simulink model "OpenLoop_TraditionalStepper"  (R2026a)
settings: Solver=FixedStepDiscrete  StopTime=0.05  FixedStep=Ts_sim
undefined symbols (not defined in the file): adc_counts_at_zero_current, amps_per_adc_count, number_of_steps_to_move, phase_voltage_volts, sequence_start_angle_radians, step_angle_radians, step_direction, step_rate_steps_per_second, step_sequence_phase_a, step_sequence_phase_b, steps_in_sequence, Ts_sim
settings Model: Creator=drew  LastModifiedBy=Drew

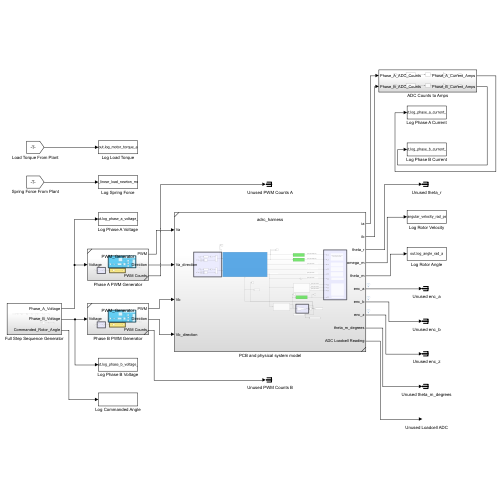
[thumbnail: Simulink's stored preview of the top-level diagram]
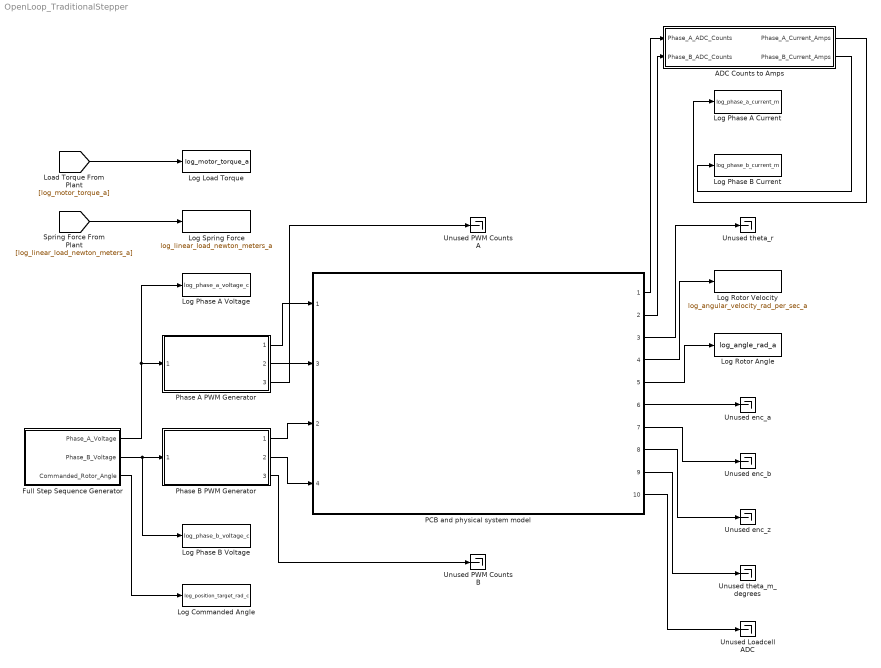
== system OpenLoop_TraditionalStepper ==
  ADC Counts to Amps : Subsystem
  Full Step Sequence Generator : Subsystem
  Log Commanded Angle : ToWorkspace  VariableName=log_position_target_rad_c  SaveFormat=Timeseries  SampleTime=-1
      settings: Decimation=logging_decimation
  Log Load Torque : ToWorkspace  VariableName=log_motor_torque_a  SaveFormat=Timeseries  SampleTime=-1
      settings: Decimation=logging_decimation
  Log Phase A Current : ToWorkspace  VariableName=log_phase_a_current_m  SaveFormat=Timeseries  SampleTime=-1
      settings: Decimation=logging_decimation
  Log Phase A Voltage : ToWorkspace  VariableName=log_phase_a_voltage_c  SaveFormat=Timeseries  SampleTime=-1
      settings: Decimation=logging_decimation
  Log Phase B Current : ToWorkspace  VariableName=log_phase_b_current_m  SaveFormat=Timeseries  SampleTime=-1
      settings: Decimation=logging_decimation
  Log Phase B Voltage : ToWorkspace  VariableName=log_phase_b_voltage_c  SaveFormat=Timeseries  SampleTime=-1
      settings: Decimation=logging_decimation
  Log Rotor Angle : ToWorkspace  VariableName=log_angle_rad_a  SaveFormat=Timeseries  SampleTime=-1
      settings: Decimation=logging_decimation
  Log Rotor Velocity : ToWorkspace  VariableName=log_angular_velocity_rad_per_sec_a  SaveFormat=Timeseries  SampleTime=-1
      settings: Decimation=logging_decimation
  Log Spring Force : ToWorkspace  VariableName=log_linear_load_newton_meters_a  SaveFormat=Timeseries  SampleTime=-1
      settings: Decimation=logging_decimation
  PCB and physical system model : Subsystem  ReferencedSubsystem=adrc_harness
      settings: PortSchema="{\"entries\":[{\"content\":{\"sides\":[{\"content\":{\"connectorIds\":[\"In1\",\"In3\",\"In2\",\"In4\"]},\"type\":\"ConnectorPlacement.EquallySpacedRectSide\",\"uuid\":\"db952c66-fc57-447a-862c-b79330cada38\"},{\"content\":{\"connectorIds\":[\"Out1\",\"Out2\",\"Out3\",\"Out4\",\"Out5\",\"Out6\",\"Out7\",\"Out8\",\"Out9\",\"Out10\"],\"side\":\"RIGHT\"},\"type\":\"ConnectorPlacement.EquallySpacedRectSide\",\"uuid\":\"12562dc1-b5c4-4239-b729-963395de8428\"},{\"content\":{\"side\":\"TOP\"},\"type\":\"ConnectorPlacement.EquallySpacedRectSide\",\"uuid\":\"3dbdfbee-8cdb-483e-891a-ab3c030ef055\"}]},\"type\":\"ConnectorPlacement.EquallySpacedConnector\",\"uuid\":\"9d79cb43-5fdf-4c5b-b972-7a6fb554b8ba\"}],\"packageUris\":[\"http://schema.mathworks.com/mf0/Connector/R2020b\"],\"version\":\"1.0\"}"
  Phase A PWM Generator : Subsystem  ReferencedSubsystem=PWM_Generator
  Phase B PWM Generator : Subsystem  ReferencedSubsystem=PWM_Generator
  Unused Loadcell ADC : Terminator
  Unused PWM Counts A : Terminator
  Unused PWM Counts B : Terminator
  Unused enc_a : Terminator
  Unused enc_b : Terminator
  Unused enc_z : Terminator
  Unused theta_m_degrees : Terminator
  Unused theta_r : Terminator
  wires:
  Phase B PWM Generator/3 -> Unused PWM Counts B/1
  Phase A PWM Generator/3 -> Unused PWM Counts A/1
  PCB and physical system model/10 -> Unused Loadcell ADC/1
  PCB and physical system model/9 -> Unused theta_m_degrees/1
  PCB and physical system model/8 -> Unused enc_z/1
  PCB and physical system model/7 -> Unused enc_b/1
  PCB and physical system model/6 -> Unused enc_a/1
  PCB and physical system model/3 -> Unused theta_r/1
  [log_linear_load_newton_meters_a] -> Log Spring Force/1
  [log_motor_torque_a] -> Log Load Torque/1
  PCB and physical system model/5 -> Log Rotor Angle/1
  PCB and physical system model/4 -> Log Rotor Velocity/1
  Full Step Sequence Generator/3(Commanded_Rotor_Angle) -> Log Commanded Angle/1
  Full Step Sequence Generator/1(Phase_A_Voltage) -> Phase A PWM Generator/1, Log Phase A Voltage/1
  Full Step Sequence Generator/2(Phase_B_Voltage) -> Phase B PWM Generator/1, Log Phase B Voltage/1
  Phase B PWM Generator/2 -> PCB and physical system model/4
  Phase B PWM Generator/1 -> PCB and physical system model/2
  Phase A PWM Generator/2 -> PCB and physical system model/3
  Phase A PWM Generator/1 -> PCB and physical system model/1
  ADC Counts to Amps/2(Phase_B_Current_Amps) -> Log Phase B Current/1
  ADC Counts to Amps/1(Phase_A_Current_Amps) -> Log Phase A Current/1
  PCB and physical system model/1 -> ADC Counts to Amps/1(Phase_A_ADC_Counts)
  PCB and physical system model/2 -> ADC Counts to Amps/2(Phase_B_ADC_Counts)

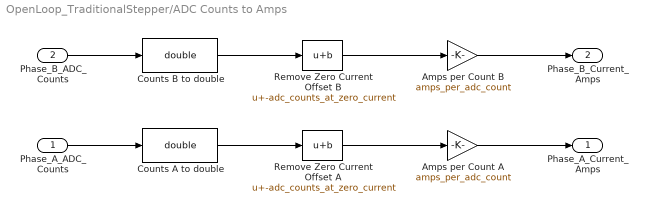
== system OpenLoop_TraditionalStepper/ADC Counts to Amps ==
  Phase_A_ADC_Counts : Inport
  Phase_B_ADC_Counts : Inport  Port=2
  Amps per Count A : Gain  Gain=amps_per_adc_count
  Amps per Count B : Gain  Gain=amps_per_adc_count
  Counts A to double : DataTypeConversion  OutDataTypeStr=double  SaturateOnIntegerOverflow=off  RndMeth=Floor
  Counts B to double : DataTypeConversion  OutDataTypeStr=double  SaturateOnIntegerOverflow=off  RndMeth=Floor
  Remove Zero Current Offset A : Bias  Bias=-adc_counts_at_zero_current  SaturateOnIntegerOverflow=off
  Remove Zero Current Offset B : Bias  Bias=-adc_counts_at_zero_current  SaturateOnIntegerOverflow=off
  Phase_A_Current_Amps : Outport
  Phase_B_Current_Amps : Outport  Port=2
  wires:
  Amps per Count B/1 -> Phase_B_Current_Amps/1
  Remove Zero Current Offset B/1 -> Amps per Count B/1
  Counts B to double/1 -> Remove Zero Current Offset B/1
  Phase_B_ADC_Counts/1 -> Counts B to double/1
  Amps per Count A/1 -> Phase_A_Current_Amps/1
  Remove Zero Current Offset A/1 -> Amps per Count A/1
  Counts A to double/1 -> Remove Zero Current Offset A/1
  Phase_A_ADC_Counts/1 -> Counts A to double/1

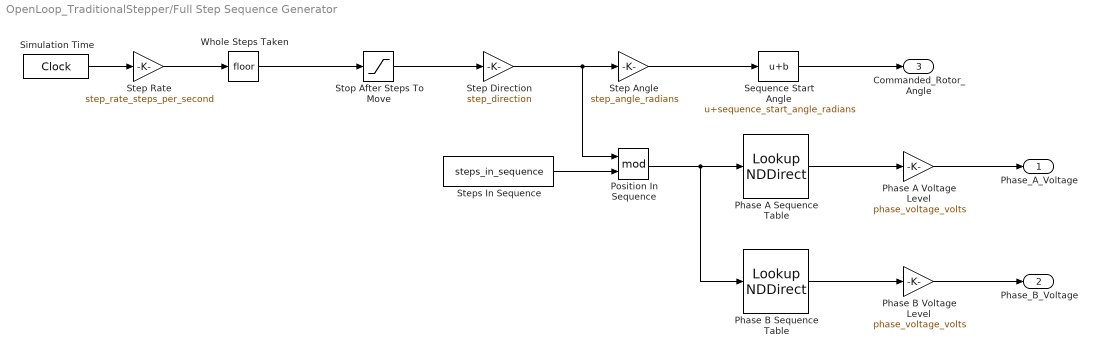
== system OpenLoop_TraditionalStepper/Full Step Sequence Generator ==
  Phase A Sequence Table : LookupNDDirect  NumberOfTableDimensions=1  Table=step_sequence_phase_a
  Phase A Voltage Level : Gain  Gain=phase_voltage_volts
  Phase B Sequence Table : LookupNDDirect  NumberOfTableDimensions=1  Table=step_sequence_phase_b
  Phase B Voltage Level : Gain  Gain=phase_voltage_volts
  Position In Sequence : Math  Operator=mod
  Sequence Start Angle : Bias  Bias=sequence_start_angle_radians  SaturateOnIntegerOverflow=off
  Simulation Time : DigitalClock  SampleTime=Ts_sim
  Step Angle : Gain  Gain=step_angle_radians
  Step Direction : Gain  Gain=step_direction
  Step Rate : Gain  Gain=step_rate_steps_per_second
  Steps In Sequence : Constant  Value=steps_in_sequence
  Stop After Steps To Move : Saturate  UpperLimit=number_of_steps_to_move  LowerLimit=0
  Whole Steps Taken : Rounding
  Phase_A_Voltage : Outport
  Phase_B_Voltage : Outport  Port=2
  Commanded_Rotor_Angle : Outport  Port=3
  wires:
  Stop After Steps To Move/1 -> Step Direction/1
  Whole Steps Taken/1 -> Stop After Steps To Move/1
  Step Rate/1 -> Whole Steps Taken/1
  Simulation Time/1 -> Step Rate/1
  Sequence Start Angle/1 -> Commanded_Rotor_Angle/1
  Step Direction/1 -> Step Angle/1, Position In Sequence/1
  Steps In Sequence/1 -> Position In Sequence/2
  Position In Sequence/1 -> Phase B Sequence Table/1, Phase A Sequence Table/1
  Phase A Sequence Table/1 -> Phase A Voltage Level/1
  Phase B Sequence Table/1 -> Phase B Voltage Level/1
  Phase A Voltage Level/1 -> Phase_A_Voltage/1
  Phase B Voltage Level/1 -> Phase_B_Voltage/1
  Step Angle/1 -> Sequence Start Angle/1
